simulink model "DDMR_Simscape_PID_Motor_HBridge"  (R2024b)
settings: Solver=ode23t  StartTime=0.0  StopTime=30  FixedStep=0.005  RelTol=1e-3
values from neighbouring files (symbols this model uses):
  L = 0.2    [LQR.m]    (also in Track.m; Track2.m)
  L_f = 0.2    [LQR.m]    (also in Track.m; Track2.m)
  line_width = 0.03    [LQR.m]    (also in Track.m; Track2.m)
  N = size(pts, 1)    [Track2.m]
  R = 0.05    [LQR.m]    (also in Track.m; Track2.m)
  track_pts = [2*cos(linspace(0, 2*pi, 1000)'), 2*sin(linspace(0, 2*pi, 1000)').*cos(linspace(0, 2*pi, 1000)')]    [LQR.m]    (also in Track.m; Track2.m = [track_pts; segments{i}])
  W_spread = 0.15    [LQR.m]    (also in Track.m; Track2.m)
undefined symbols (not defined in the file or in its folder): X, Y, Z
libraries: sm_lib x22, fl_lib x15, nesl_utility x10, ee_lib x6, slpidlib x4, simulink x2, batteryecm_lib x1
(part 2 of 2)

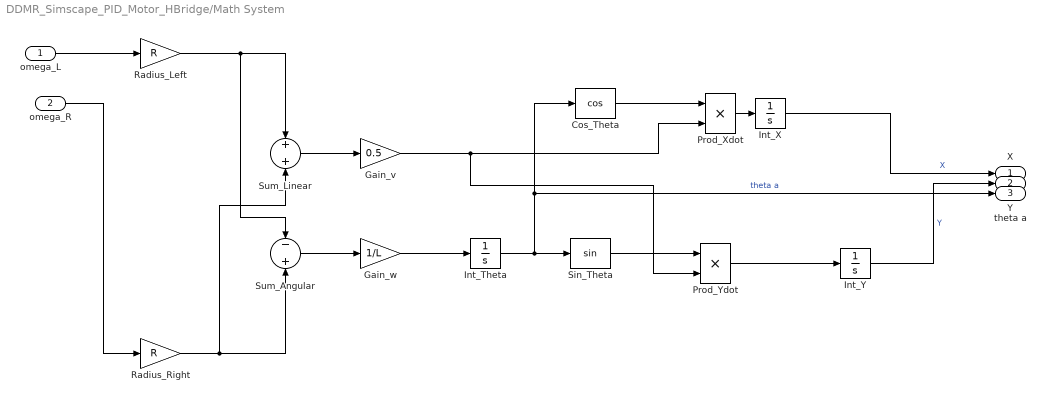
== system DDMR_Simscape_PID_Motor_HBridge/Math System ==
  omega_L : Inport
  omega_R : Inport  Port=2
  Cos_Theta : Trigonometry  Operator=cos
  Gain_v : Gain  Gain=0.5
  Gain_w : Gain  Gain=1/L
  Int_Theta : Integrator  InitialCondition=pi/-3
  Int_X : Integrator
  Int_Y : Integrator
  Prod_Xdot : Product
  Prod_Ydot : Product
  Radius_Left : Gain  Gain=R
  Radius_Right : Gain  Gain=R
  Sin_Theta : Trigonometry
  Sum_Angular : Sum  Inputs=-+
  Sum_Linear : Sum
  X : Outport
  Y : Outport  Port=2
  theta a : Outport  Port=3
  wires:
  Radius_Right/1 -> Sum_Linear/2, Sum_Angular/2
  Radius_Left/1 -> Sum_Linear/1, Sum_Angular/1
  Int_Y/1 -> Y/1  "Y"
  Prod_Ydot/1 -> Int_Y/1
  Gain_v/1 -> Prod_Xdot/2, Prod_Ydot/2
  Sum_Angular/1 -> Gain_w/1
  Int_Theta/1 -> theta a/1, Cos_Theta/1, Sin_Theta/1  "theta a"
  Sum_Linear/1 -> Gain_v/1
  Cos_Theta/1 -> Prod_Xdot/1
  Gain_w/1 -> Int_Theta/1
  Prod_Xdot/1 -> Int_X/1
  Sin_Theta/1 -> Prod_Ydot/1
  omega_R/1 -> Radius_Right/1
  omega_L/1 -> Radius_Left/1
  Int_X/1 -> X/1  "X"

== matlab function DDMR_Simscape_PID_Motor_HBridge/6-Sensor Array1 ==
  data: x input; sensor_readings output; y input; theta input; track_pts input; L_f input; W_spread input; threshold input; sensor_pos output
function [sensor_readings, sensor_pos] = fcn(x, y, theta, track_pts, L_f, W_spread, threshold)
    % 6 sensors spread linearly across the front
    y_offsets = linspace(W_spread/2, -W_spread/2, 6);
    S_loc = [L_f * ones(1,6); y_offsets];
    
    R = [cos(theta), -sin(theta); sin(theta), cos(theta)];
    
    sensor_pos = zeros(2, 6);
    sensor_readings = zeros(1, 6);
    
    for i = 1:6
        % Calculate global position of each sensor
        sensor_pos(:, i) = [x; y] + R * S_loc(:, i);
        
        % Check distance to the track
        dists = sqrt((track_pts(:,1) - sensor_pos(1, i)).^2 + (track_pts(:,2) - sensor_pos(2, i)).^2);
        if min(dists) <= threshold
            sensor_readings(i) = 1;
        end
    end
end

== matlab function DDMR_Simscape_PID_Motor_HBridge/Inverse_Kinematiks 1 ==
  data: v input; omega_L output; omega input; R input; L input; omega_R output
function [omega_L, omega_R] = inverse_kinematics(v, omega, R, L)
    % Calculate linear velocity of each wheel (m/s)
    v_L = v - (omega * L / 2);
    v_R = v + (omega * L / 2);

    % Convert linear velocity to angular velocity (rad/s)
    omega_L = v_L / R;
    omega_R = v_R / R;
end

== matlab function DDMR_Simscape_PID_Motor_HBridge/MATLAB Function1 ==
  settings: updateMethod=DISCRETE
  data: sensor_readings input; error output
function error = calculate_error(sensor_readings)
    % Physical spatial weights mapped to the 6-sensor array. 
    % Far left is positive, far right is negative to match original steering convention.
    weights = [2.5, 1.5, 0.5, -0.5, -1.5, -2.5]; 
    
    persistent prev_error;
    if isempty(prev_error)
        prev_error = 0;
    end
    
    % Determine how many sensors currently see the line
    active_sensors = sum(sensor_readings);
    
    if active_sensors == 0
        % Track lost: rely on memory to keep steering back toward the line
        error = prev_error; 
    else
        % Track found: Calculate the continuous center of mass (centroid)
        error = sum(sensor_readings .* weights) / active_sensors;
        prev_error = error; 
    end
end
